simulink model "untitled"  (R2025b)
settings: Solver=ode1be  StartTime=0.0  StopTime=15  FixedStep=0.001  RelTol=1e-3
undefined symbols (not defined in the file): DiscIntNeverNeededParam, X, Y, Z
libraries: sm_lib x94, nesl_utility x30, fl_lib x14, ee_lib x5, simulink_extras x4, instrumentseriallib x4, etargetslib x3
(part 3 of 4)

== system untitled/Subsystem1/시스템 응답특성 ==
  MATLAB Function : MATLAB Function  TreatAsAtomicUnit=on
  감쇠비 : Display
  감쇠진동수 : Display
  고유진동수 : Display
  정착시간 : Display
  진동횟수 : Display
  wires:
  MATLAB Function/1(wn) -> 고유진동수/1
  MATLAB Function/3(wd) -> 감쇠진동수/1
  MATLAB Function/4(ts) -> 정착시간/1
  MATLAB Function/2(zeta) -> 감쇠비/1
  [cal_d] -> MATLAB Function/2(kd)
  [cal_p] -> MATLAB Function/1(kp)
  MATLAB Function/5(N) -> 진동횟수/1

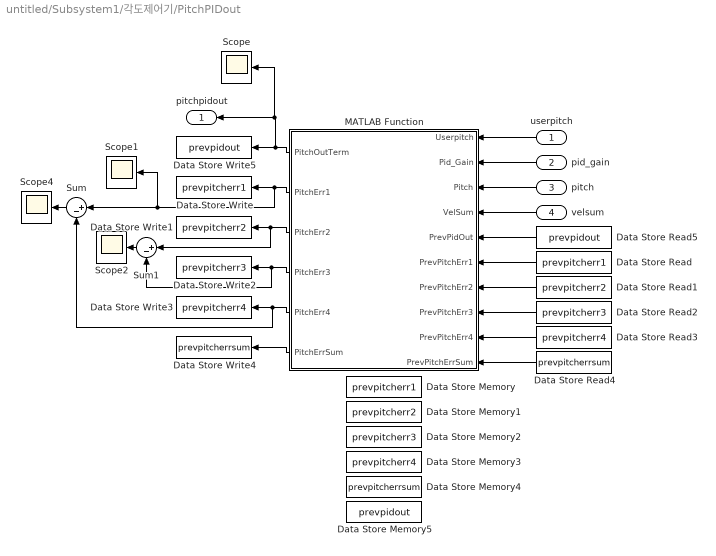
== system untitled/Subsystem1/각도제어기/PitchPIDout ==
  userpitch : Inport
  pid_gain : Inport  Port=2
  pitch : Inport  Port=3
  velsum : Inport  Port=4
  Data Store Memory : DataStoreMemory  DataStoreName=prevpitcherr1  WriteAfterWriteMsg=warning  ShowAdditionalParam=off
  Data Store Memory1 : DataStoreMemory  DataStoreName=prevpitcherr2  WriteAfterWriteMsg=warning  ShowAdditionalParam=off
  Data Store Memory2 : DataStoreMemory  DataStoreName=prevpitcherr3  WriteAfterWriteMsg=warning  ShowAdditionalParam=off
  Data Store Memory3 : DataStoreMemory  DataStoreName=prevpitcherr4  WriteAfterWriteMsg=warning  ShowAdditionalParam=off
  Data Store Memory4 : DataStoreMemory  DataStoreName=prevpitcherrsum  WriteAfterWriteMsg=warning  ShowAdditionalParam=off
  Data Store Memory5 : DataStoreMemory  DataStoreName=prevpidout  WriteAfterWriteMsg=warning  ShowAdditionalParam=off
  Data Store Read : DataStoreRead  DataStoreName=prevpitcherr1  IndexOptions=Index vector (dialog)  Indices=1  OutputSizes=1
  Data Store Read1 : DataStoreRead  DataStoreName=prevpitcherr2  IndexOptions=Index vector (dialog)  Indices=1  OutputSizes=1
  Data Store Read2 : DataStoreRead  DataStoreName=prevpitcherr3  IndexOptions=Index vector (dialog)  Indices=1  OutputSizes=1
  Data Store Read3 : DataStoreRead  DataStoreName=prevpitcherr4  IndexOptions=Index vector (dialog)  Indices=1  OutputSizes=1
  Data Store Read4 : DataStoreRead  DataStoreName=prevpitcherrsum  IndexOptions=Index vector (dialog)  Indices=1  OutputSizes=1
  Data Store Read5 : DataStoreRead  DataStoreName=prevpidout  IndexOptions=Index vector (dialog)  Indices=1  OutputSizes=1
  Data Store Write : DataStoreWrite  DataStoreName=prevpitcherr1  IndexOptions=Index vector (dialog)  Indices=1  OutputSizes=1
  Data Store Write1 : DataStoreWrite  DataStoreName=prevpitcherr2  IndexOptions=Index vector (dialog)  Indices=1  OutputSizes=1
  Data Store Write2 : DataStoreWrite  DataStoreName=prevpitcherr3  IndexOptions=Index vector (dialog)  Indices=1  OutputSizes=1
  Data Store Write3 : DataStoreWrite  DataStoreName=prevpitcherr4  IndexOptions=Index vector (dialog)  Indices=1  OutputSizes=1
  Data Store Write4 : DataStoreWrite  DataStoreName=prevpitcherrsum  IndexOptions=Index vector (dialog)  Indices=1  OutputSizes=1
  Data Store Write5 : DataStoreWrite  DataStoreName=prevpidout  IndexOptions=Index vector (dialog)  Indices=1  OutputSizes=1
  MATLAB Function : MATLAB Function  TreatAsAtomicUnit=on  SystemSampleTime=0.005
  Scope{,1..2,4} (4 alike) : Scope
      Scope settings: ActiveDisplayYMinimum=-0.020953586841830588  ActiveDisplayYMaximum=0.0054385268449779461  DataLoggingVariableName=ScopeData11
      Scope1 settings: ActiveDisplayYMinimum=-2.5668276523074756E-6  ActiveDisplayYMaximum=2.3101448870766709E-5  DataLoggingVariableName=ScopeData22
      Scope2 settings: ActiveDisplayYMinimum=-0.0010160045575017935  ActiveDisplayYMaximum=0.0011587189479117432  DataLoggingVariableName=ScopeData23
      Scope4 settings: ActiveDisplayYMinimum=-0.0018545960529793347  ActiveDisplayYMaximum=0.0021480135673250383  DataLoggingVariableName=ScopeData25
  Sum : Sum  Inputs=|+-
  Sum1 : Sum  Inputs=|+-
  pitchpidout : Outport
  wires:
  userpitch/1 -> MATLAB Function/1(Userpitch)
  pid_gain/1 -> MATLAB Function/2(Pid_Gain)
  pitch/1 -> MATLAB Function/3(Pitch)
  velsum/1 -> MATLAB Function/4(VelSum)
  Data Store Read5/1 -> MATLAB Function/5(PrevPidOut)
  Data Store Read/1 -> MATLAB Function/6(PrevPitchErr1)
  Data Store Read1/1 -> MATLAB Function/7(PrevPitchErr2)
  Data Store Read2/1 -> MATLAB Function/8(PrevPitchErr3)
  Data Store Read3/1 -> MATLAB Function/9(PrevPitchErr4)
  Data Store Read4/1 -> MATLAB Function/10(PrevPitchErrSum)
  MATLAB Function/1(PitchOutTerm) -> Scope/1, pitchpidout/1, Data Store Write5/1
  MATLAB Function/2(PitchErr1) -> Scope1/1, Sum/1, Data Store Write/1
  MATLAB Function/6(PitchErrSum) -> Data Store Write4/1
  MATLAB Function/3(PitchErr2) -> Sum1/1, Data Store Write1/1
  MATLAB Function/4(PitchErr3) -> Sum1/2, Data Store Write2/1
  MATLAB Function/5(PitchErr4) -> Sum/2, Data Store Write3/1
  Sum/1 -> Scope4/1
  Sum1/1 -> Scope2/1

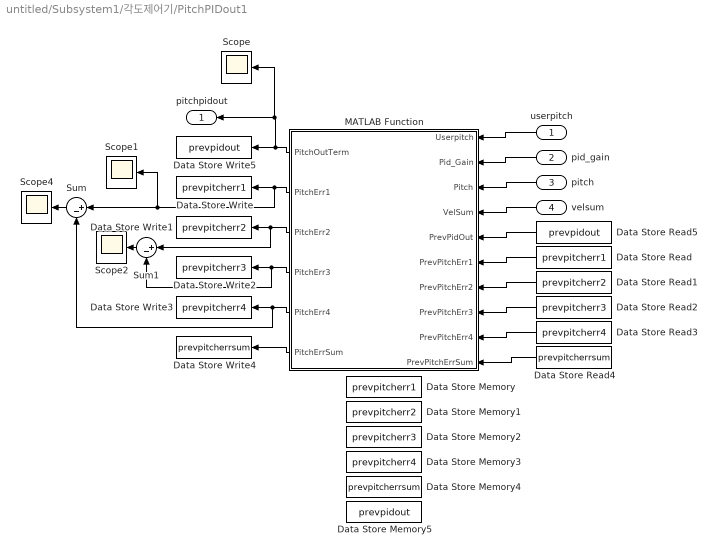
== system untitled/Subsystem1/각도제어기/PitchPIDout1 ==
  userpitch : Inport
  pid_gain : Inport  Port=2
  pitch : Inport  Port=3
  velsum : Inport  Port=4
  Data Store Memory : DataStoreMemory  DataStoreName=prevpitcherr1  WriteAfterWriteMsg=warning  ShowAdditionalParam=off
  Data Store Memory1 : DataStoreMemory  DataStoreName=prevpitcherr2  WriteAfterWriteMsg=warning  ShowAdditionalParam=off
  Data Store Memory2 : DataStoreMemory  DataStoreName=prevpitcherr3  WriteAfterWriteMsg=warning  ShowAdditionalParam=off
  Data Store Memory3 : DataStoreMemory  DataStoreName=prevpitcherr4  WriteAfterWriteMsg=warning  ShowAdditionalParam=off
  Data Store Memory4 : DataStoreMemory  DataStoreName=prevpitcherrsum  WriteAfterWriteMsg=warning  ShowAdditionalParam=off
  Data Store Memory5 : DataStoreMemory  DataStoreName=prevpidout  WriteAfterWriteMsg=warning  ShowAdditionalParam=off
  Data Store Read : DataStoreRead  DataStoreName=prevpitcherr1  IndexOptions=Index vector (dialog)  Indices=1  OutputSizes=1
  Data Store Read1 : DataStoreRead  DataStoreName=prevpitcherr2  IndexOptions=Index vector (dialog)  Indices=1  OutputSizes=1
  Data Store Read2 : DataStoreRead  DataStoreName=prevpitcherr3  IndexOptions=Index vector (dialog)  Indices=1  OutputSizes=1
  Data Store Read3 : DataStoreRead  DataStoreName=prevpitcherr4  IndexOptions=Index vector (dialog)  Indices=1  OutputSizes=1
  Data Store Read4 : DataStoreRead  DataStoreName=prevpitcherrsum  IndexOptions=Index vector (dialog)  Indices=1  OutputSizes=1
  Data Store Read5 : DataStoreRead  DataStoreName=prevpidout  IndexOptions=Index vector (dialog)  Indices=1  OutputSizes=1
  Data Store Write : DataStoreWrite  DataStoreName=prevpitcherr1  IndexOptions=Index vector (dialog)  Indices=1  OutputSizes=1
  Data Store Write1 : DataStoreWrite  DataStoreName=prevpitcherr2  IndexOptions=Index vector (dialog)  Indices=1  OutputSizes=1
  Data Store Write2 : DataStoreWrite  DataStoreName=prevpitcherr3  IndexOptions=Index vector (dialog)  Indices=1  OutputSizes=1
  Data Store Write3 : DataStoreWrite  DataStoreName=prevpitcherr4  IndexOptions=Index vector (dialog)  Indices=1  OutputSizes=1
  Data Store Write4 : DataStoreWrite  DataStoreName=prevpitcherrsum  IndexOptions=Index vector (dialog)  Indices=1  OutputSizes=1
  Data Store Write5 : DataStoreWrite  DataStoreName=prevpidout  IndexOptions=Index vector (dialog)  Indices=1  OutputSizes=1
  MATLAB Function : MATLAB Function  TreatAsAtomicUnit=on  SystemSampleTime=0.005
  Scope{,1..2,4} (4 alike) : Scope
      Scope settings: ActiveDisplayYMinimum=-0.020953586841830588  ActiveDisplayYMaximum=0.0054385268449779461  DataLoggingVariableName=ScopeData11
      Scope1 settings: ActiveDisplayYMinimum=-2.5668276523074756E-6  ActiveDisplayYMaximum=2.3101448870766709E-5  DataLoggingVariableName=ScopeData22
      Scope2 settings: ActiveDisplayYMinimum=-0.0010160045575017935  ActiveDisplayYMaximum=0.0011587189479117432  DataLoggingVariableName=ScopeData23
      Scope4 settings: ActiveDisplayYMinimum=-0.0018545960529793347  ActiveDisplayYMaximum=0.0021480135673250383  DataLoggingVariableName=ScopeData25
  Sum : Sum  Inputs=|+-
  Sum1 : Sum  Inputs=|+-
  pitchpidout : Outport
  wires:
  userpitch/1 -> MATLAB Function/1(Userpitch)
  pid_gain/1 -> MATLAB Function/2(Pid_Gain)
  pitch/1 -> MATLAB Function/3(Pitch)
  velsum/1 -> MATLAB Function/4(VelSum)
  Data Store Read5/1 -> MATLAB Function/5(PrevPidOut)
  Data Store Read/1 -> MATLAB Function/6(PrevPitchErr1)
  Data Store Read1/1 -> MATLAB Function/7(PrevPitchErr2)
  Data Store Read2/1 -> MATLAB Function/8(PrevPitchErr3)
  Data Store Read3/1 -> MATLAB Function/9(PrevPitchErr4)
  Data Store Read4/1 -> MATLAB Function/10(PrevPitchErrSum)
  MATLAB Function/1(PitchOutTerm) -> Scope/1, pitchpidout/1, Data Store Write5/1
  MATLAB Function/2(PitchErr1) -> Scope1/1, Sum/1, Data Store Write/1
  MATLAB Function/6(PitchErrSum) -> Data Store Write4/1
  MATLAB Function/3(PitchErr2) -> Sum1/1, Data Store Write1/1
  MATLAB Function/4(PitchErr3) -> Sum1/2, Data Store Write2/1
  MATLAB Function/5(PitchErr4) -> Sum/2, Data Store Write3/1
  Sum/1 -> Scope4/1
  Sum1/1 -> Scope2/1

== system untitled/Subsystem1/각도제어기/TargetPIDout ==
  TargetVel : Inport
  robot_vel : Inport  Port=2
  pid_gain : Inport  Port=3
  Data Store Memory : DataStoreMemory  DataStoreName=prevTargeterr1  WriteAfterWriteMsg=warning  ShowAdditionalParam=off
  Data Store Memory1 : DataStoreMemory  DataStoreName=prevTargeterr2  WriteAfterWriteMsg=warning  ShowAdditionalParam=off
  Data Store Memory2 : DataStoreMemory  DataStoreName=prevTargeterr3  WriteAfterWriteMsg=warning  ShowAdditionalParam=off
  Data Store Memory3 : DataStoreMemory  DataStoreName=prevTargeterr4  WriteAfterWriteMsg=warning  ShowAdditionalParam=off
  Data Store Memory4 : DataStoreMemory  DataStoreName=prevTargetErrSum  WriteAfterWriteMsg=warning  ShowAdditionalParam=off
  Data Store Memory5 : DataStoreMemory  DataStoreName=Prevpidout  WriteAfterWriteMsg=warning  ShowAdditionalParam=off
  Data Store Read : DataStoreRead  DataStoreName=prevTargeterr1  IndexOptions=Index vector (dialog)  Indices=1  OutputSizes=1
  Data Store Read1 : DataStoreRead  DataStoreName=prevTargeterr2  IndexOptions=Index vector (dialog)  Indices=1  OutputSizes=1
  Data Store Read2 : DataStoreRead  DataStoreName=prevTargeterr3  IndexOptions=Index vector (dialog)  Indices=1  OutputSizes=1
  Data Store Read3 : DataStoreRead  DataStoreName=prevTargeterr4  IndexOptions=Index vector (dialog)  Indices=1  OutputSizes=1
  Data Store Read4 : DataStoreRead  DataStoreName=prevTargetErrSum  IndexOptions=Index vector (dialog)  Indices=1  OutputSizes=1
  Data Store Read5 : DataStoreRead  DataStoreName=Prevpidout  IndexOptions=Index vector (dialog)  Indices=1  OutputSizes=1
  Data Store Write : DataStoreWrite  DataStoreName=prevTargeterr1  IndexOptions=Index vector (dialog)  Indices=1  OutputSizes=1
  Data Store Write1 : DataStoreWrite  DataStoreName=prevTargeterr2  IndexOptions=Index vector (dialog)  Indices=1  OutputSizes=1
  Data Store Write2 : DataStoreWrite  DataStoreName=prevTargeterr3  IndexOptions=Index vector (dialog)  Indices=1  OutputSizes=1
  Data Store Write3 : DataStoreWrite  DataStoreName=prevTargeterr4  IndexOptions=Index vector (dialog)  Indices=1  OutputSizes=1
  Data Store Write4 : DataStoreWrite  DataStoreName=prevTargetErrSum  IndexOptions=Index vector (dialog)  Indices=1  OutputSizes=1
  Data Store Write5 : DataStoreWrite  DataStoreName=Prevpidout  IndexOptions=Index vector (dialog)  Indices=1  OutputSizes=1
  MATLAB Function : MATLAB Function  TreatAsAtomicUnit=on  SystemSampleTime=0.005
  UserPitch : Outport
  wires:
  Data Store Read5/1 -> MATLAB Function/4(PrevPidOut)
  MATLAB Function/6(TargetErrSum) -> Data Store Write4/1
  Data Store Read3/1 -> MATLAB Function/8(PrevTargetErr4)
  MATLAB Function/4(TargetErr3) -> Data Store Write2/1
  Data Store Read1/1 -> MATLAB Function/6(PrevTargetErr2)
  MATLAB Function/2(TargetErr1) -> Data Store Write/1
  Data Store Read4/1 -> MATLAB Function/9(PrevYawErrSum)
  Data Store Read2/1 -> MATLAB Function/7(PrevTargetErr3)
  pid_gain/1 -> MATLAB Function/3(Pid_Gain)
  MATLAB Function/1(UserPitch) -> UserPitch/1, Data Store Write5/1
  MATLAB Function/3(TargetErr2) -> Data Store Write1/1
  Data Store Read/1 -> MATLAB Function/5(PrevTargetErr1)
  TargetVel/1 -> MATLAB Function/1(TargetVel)
  MATLAB Function/5(TargetErr4) -> Data Store Write3/1
  robot_vel/1 -> MATLAB Function/2(robot_vel)

== system untitled/Subsystem1/각도제어기/TargetPIDout1 ==
  TargetVel : Inport
  robot_vel : Inport  Port=2
  pid_gain : Inport  Port=3
  Data Store Memory : DataStoreMemory  DataStoreName=prevTargeterr1  WriteAfterWriteMsg=warning  ShowAdditionalParam=off
  Data Store Memory1 : DataStoreMemory  DataStoreName=prevTargeterr2  WriteAfterWriteMsg=warning  ShowAdditionalParam=off
  Data Store Memory2 : DataStoreMemory  DataStoreName=prevTargeterr3  WriteAfterWriteMsg=warning  ShowAdditionalParam=off
  Data Store Memory3 : DataStoreMemory  DataStoreName=prevTargeterr4  WriteAfterWriteMsg=warning  ShowAdditionalParam=off
  Data Store Memory4 : DataStoreMemory  DataStoreName=prevTargetErrSum  WriteAfterWriteMsg=warning  ShowAdditionalParam=off
  Data Store Memory5 : DataStoreMemory  DataStoreName=Prevpidout  WriteAfterWriteMsg=warning  ShowAdditionalParam=off
  Data Store Read : DataStoreRead  DataStoreName=prevTargeterr1  IndexOptions=Index vector (dialog)  Indices=1  OutputSizes=1
  Data Store Read1 : DataStoreRead  DataStoreName=prevTargeterr2  IndexOptions=Index vector (dialog)  Indices=1  OutputSizes=1
  Data Store Read2 : DataStoreRead  DataStoreName=prevTargeterr3  IndexOptions=Index vector (dialog)  Indices=1  OutputSizes=1
  Data Store Read3 : DataStoreRead  DataStoreName=prevTargeterr4  IndexOptions=Index vector (dialog)  Indices=1  OutputSizes=1
  Data Store Read4 : DataStoreRead  DataStoreName=prevTargetErrSum  IndexOptions=Index vector (dialog)  Indices=1  OutputSizes=1
  Data Store Read5 : DataStoreRead  DataStoreName=Prevpidout  IndexOptions=Index vector (dialog)  Indices=1  OutputSizes=1
  Data Store Write : DataStoreWrite  DataStoreName=prevTargeterr1  IndexOptions=Index vector (dialog)  Indices=1  OutputSizes=1
  Data Store Write1 : DataStoreWrite  DataStoreName=prevTargeterr2  IndexOptions=Index vector (dialog)  Indices=1  OutputSizes=1
  Data Store Write2 : DataStoreWrite  DataStoreName=prevTargeterr3  IndexOptions=Index vector (dialog)  Indices=1  OutputSizes=1
  Data Store Write3 : DataStoreWrite  DataStoreName=prevTargeterr4  IndexOptions=Index vector (dialog)  Indices=1  OutputSizes=1
  Data Store Write4 : DataStoreWrite  DataStoreName=prevTargetErrSum  IndexOptions=Index vector (dialog)  Indices=1  OutputSizes=1
  Data Store Write5 : DataStoreWrite  DataStoreName=Prevpidout  IndexOptions=Index vector (dialog)  Indices=1  OutputSizes=1
  MATLAB Function : MATLAB Function  TreatAsAtomicUnit=on  SystemSampleTime=0.005
  UserPitch : Outport
  wires:
  Data Store Read5/1 -> MATLAB Function/4(PrevPidOut)
  MATLAB Function/6(TargetErrSum) -> Data Store Write4/1
  Data Store Read3/1 -> MATLAB Function/8(PrevTargetErr4)
  MATLAB Function/4(TargetErr3) -> Data Store Write2/1
  Data Store Read1/1 -> MATLAB Function/6(PrevTargetErr2)
  MATLAB Function/2(TargetErr1) -> Data Store Write/1
  Data Store Read4/1 -> MATLAB Function/9(PrevYawErrSum)
  Data Store Read2/1 -> MATLAB Function/7(PrevTargetErr3)
  pid_gain/1 -> MATLAB Function/3(Pid_Gain)
  MATLAB Function/1(UserPitch) -> UserPitch/1, Data Store Write5/1
  MATLAB Function/3(TargetErr2) -> Data Store Write1/1
  Data Store Read/1 -> MATLAB Function/5(PrevTargetErr1)
  TargetVel/1 -> MATLAB Function/1(TargetVel)
  MATLAB Function/5(TargetErr4) -> Data Store Write3/1
  robot_vel/1 -> MATLAB Function/2(robot_vel)

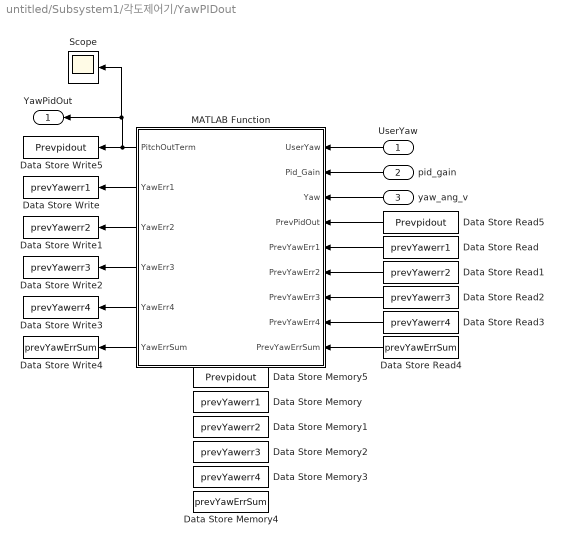
== system untitled/Subsystem1/각도제어기/YawPIDout ==
  UserYaw : Inport
  pid_gain : Inport  Port=2
  yaw_ang_v : Inport  Port=3
  Data Store Memory : DataStoreMemory  DataStoreName=prevYawerr1  WriteAfterWriteMsg=warning  ShowAdditionalParam=off
  Data Store Memory1 : DataStoreMemory  DataStoreName=prevYawerr2  WriteAfterWriteMsg=warning  ShowAdditionalParam=off
  Data Store Memory2 : DataStoreMemory  DataStoreName=prevYawerr3  WriteAfterWriteMsg=warning  ShowAdditionalParam=off
  Data Store Memory3 : DataStoreMemory  DataStoreName=prevYawerr4  WriteAfterWriteMsg=warning  ShowAdditionalParam=off
  Data Store Memory4 : DataStoreMemory  DataStoreName=prevYawErrSum  WriteAfterWriteMsg=warning  ShowAdditionalParam=off
  Data Store Memory5 : DataStoreMemory  DataStoreName=Prevpidout  WriteAfterWriteMsg=warning  ShowAdditionalParam=off
  Data Store Read : DataStoreRead  DataStoreName=prevYawerr1  IndexOptions=Index vector (dialog)  Indices=1  OutputSizes=1
  Data Store Read1 : DataStoreRead  DataStoreName=prevYawerr2  IndexOptions=Index vector (dialog)  Indices=1  OutputSizes=1
  Data Store Read2 : DataStoreRead  DataStoreName=prevYawerr3  IndexOptions=Index vector (dialog)  Indices=1  OutputSizes=1
  Data Store Read3 : DataStoreRead  DataStoreName=prevYawerr4  IndexOptions=Index vector (dialog)  Indices=1  OutputSizes=1
  Data Store Read4 : DataStoreRead  DataStoreName=prevYawErrSum  IndexOptions=Index vector (dialog)  Indices=1  OutputSizes=1
  Data Store Read5 : DataStoreRead  DataStoreName=Prevpidout  IndexOptions=Index vector (dialog)  Indices=1  OutputSizes=1
  Data Store Write : DataStoreWrite  DataStoreName=prevYawerr1  IndexOptions=Index vector (dialog)  Indices=1  OutputSizes=1
  Data Store Write1 : DataStoreWrite  DataStoreName=prevYawerr2  IndexOptions=Index vector (dialog)  Indices=1  OutputSizes=1
  Data Store Write2 : DataStoreWrite  DataStoreName=prevYawerr3  IndexOptions=Index vector (dialog)  Indices=1  OutputSizes=1
  Data Store Write3 : DataStoreWrite  DataStoreName=prevYawerr4  IndexOptions=Index vector (dialog)  Indices=1  OutputSizes=1
  Data Store Write4 : DataStoreWrite  DataStoreName=prevYawErrSum  IndexOptions=Index vector (dialog)  Indices=1  OutputSizes=1
  Data Store Write5 : DataStoreWrite  DataStoreName=Prevpidout  IndexOptions=Index vector (dialog)  Indices=1  OutputSizes=1
  MATLAB Function : MATLAB Function  TreatAsAtomicUnit=on  SystemSampleTime=0.005
  Scope : Scope
      settings: ActiveDisplayYMinimum=-0.13106550411433154  ActiveDisplayYMaximum=1.1795895370289842  DataLoggingVariableName=ScopeData15
  YawPidOut : Outport
  wires:
  Data Store Read5/1 -> MATLAB Function/4(PrevPidOut)
  MATLAB Function/6(YawErrSum) -> Data Store Write4/1
  Data Store Read3/1 -> MATLAB Function/8(PrevYawErr4)
  MATLAB Function/4(YawErr3) -> Data Store Write2/1
  Data Store Read1/1 -> MATLAB Function/6(PrevYawErr2)
  yaw_ang_v/1 -> MATLAB Function/3(Yaw)
  MATLAB Function/2(YawErr1) -> Data Store Write/1
  Data Store Read4/1 -> MATLAB Function/9(PrevYawErrSum)
  Data Store Read2/1 -> MATLAB Function/7(PrevYawErr3)
  pid_gain/1 -> MATLAB Function/2(Pid_Gain)
  MATLAB Function/1(PitchOutTerm) -> Scope/1, YawPidOut/1, Data Store Write5/1
  MATLAB Function/3(YawErr2) -> Data Store Write1/1
  Data Store Read/1 -> MATLAB Function/5(PrevYawErr1)
  UserYaw/1 -> MATLAB Function/1(UserYaw)
  MATLAB Function/5(YawErr4) -> Data Store Write3/1

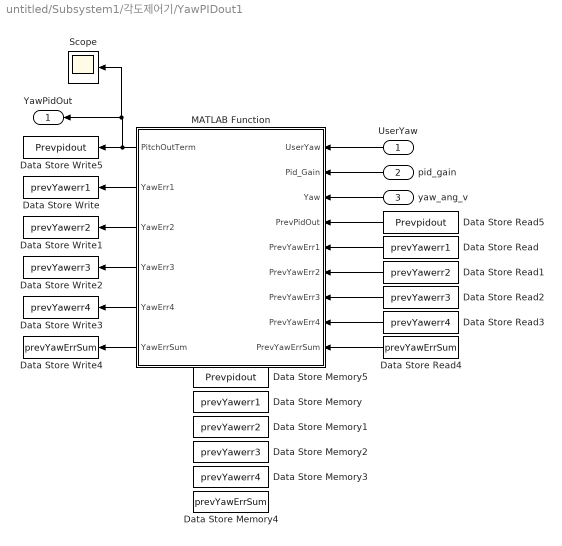
== system untitled/Subsystem1/각도제어기/YawPIDout1 ==
  UserYaw : Inport
  pid_gain : Inport  Port=2
  yaw_ang_v : Inport  Port=3
  Data Store Memory : DataStoreMemory  DataStoreName=prevYawerr1  WriteAfterWriteMsg=warning  ShowAdditionalParam=off
  Data Store Memory1 : DataStoreMemory  DataStoreName=prevYawerr2  WriteAfterWriteMsg=warning  ShowAdditionalParam=off
  Data Store Memory2 : DataStoreMemory  DataStoreName=prevYawerr3  WriteAfterWriteMsg=warning  ShowAdditionalParam=off
  Data Store Memory3 : DataStoreMemory  DataStoreName=prevYawerr4  WriteAfterWriteMsg=warning  ShowAdditionalParam=off
  Data Store Memory4 : DataStoreMemory  DataStoreName=prevYawErrSum  WriteAfterWriteMsg=warning  ShowAdditionalParam=off
  Data Store Memory5 : DataStoreMemory  DataStoreName=Prevpidout  WriteAfterWriteMsg=warning  ShowAdditionalParam=off
  Data Store Read : DataStoreRead  DataStoreName=prevYawerr1  IndexOptions=Index vector (dialog)  Indices=1  OutputSizes=1
  Data Store Read1 : DataStoreRead  DataStoreName=prevYawerr2  IndexOptions=Index vector (dialog)  Indices=1  OutputSizes=1
  Data Store Read2 : DataStoreRead  DataStoreName=prevYawerr3  IndexOptions=Index vector (dialog)  Indices=1  OutputSizes=1
  Data Store Read3 : DataStoreRead  DataStoreName=prevYawerr4  IndexOptions=Index vector (dialog)  Indices=1  OutputSizes=1
  Data Store Read4 : DataStoreRead  DataStoreName=prevYawErrSum  IndexOptions=Index vector (dialog)  Indices=1  OutputSizes=1
  Data Store Read5 : DataStoreRead  DataStoreName=Prevpidout  IndexOptions=Index vector (dialog)  Indices=1  OutputSizes=1
  Data Store Write : DataStoreWrite  DataStoreName=prevYawerr1  IndexOptions=Index vector (dialog)  Indices=1  OutputSizes=1
  Data Store Write1 : DataStoreWrite  DataStoreName=prevYawerr2  IndexOptions=Index vector (dialog)  Indices=1  OutputSizes=1
  Data Store Write2 : DataStoreWrite  DataStoreName=prevYawerr3  IndexOptions=Index vector (dialog)  Indices=1  OutputSizes=1
  Data Store Write3 : DataStoreWrite  DataStoreName=prevYawerr4  IndexOptions=Index vector (dialog)  Indices=1  OutputSizes=1
  Data Store Write4 : DataStoreWrite  DataStoreName=prevYawErrSum  IndexOptions=Index vector (dialog)  Indices=1  OutputSizes=1
  Data Store Write5 : DataStoreWrite  DataStoreName=Prevpidout  IndexOptions=Index vector (dialog)  Indices=1  OutputSizes=1
  MATLAB Function : MATLAB Function  TreatAsAtomicUnit=on  SystemSampleTime=0.005
  Scope : Scope
      settings: ActiveDisplayYMinimum=-0.13106550411433154  ActiveDisplayYMaximum=1.1795895370289842  DataLoggingVariableName=ScopeData15
  YawPidOut : Outport
  wires:
  Data Store Read5/1 -> MATLAB Function/4(PrevPidOut)
  MATLAB Function/6(YawErrSum) -> Data Store Write4/1
  Data Store Read3/1 -> MATLAB Function/8(PrevYawErr4)
  MATLAB Function/4(YawErr3) -> Data Store Write2/1
  Data Store Read1/1 -> MATLAB Function/6(PrevYawErr2)
  yaw_ang_v/1 -> MATLAB Function/3(Yaw)
  MATLAB Function/2(YawErr1) -> Data Store Write/1
  Data Store Read4/1 -> MATLAB Function/9(PrevYawErrSum)
  Data Store Read2/1 -> MATLAB Function/7(PrevYawErr3)
  pid_gain/1 -> MATLAB Function/2(Pid_Gain)
  MATLAB Function/1(PitchOutTerm) -> Scope/1, YawPidOut/1, Data Store Write5/1
  MATLAB Function/3(YawErr2) -> Data Store Write1/1
  Data Store Read/1 -> MATLAB Function/5(PrevYawErr1)
  UserYaw/1 -> MATLAB Function/1(UserYaw)
  MATLAB Function/5(YawErr4) -> Data Store Write3/1

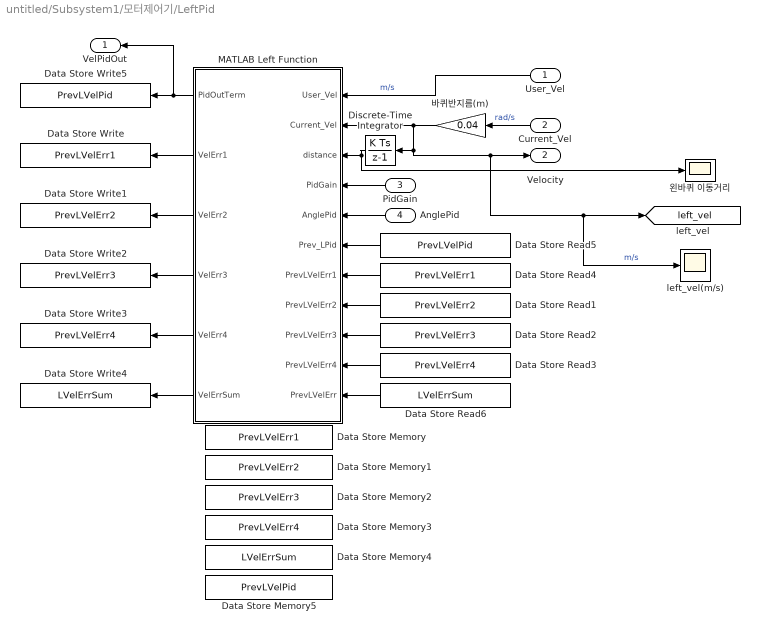
== system untitled/Subsystem1/모터제어기/LeftPid ==
  User_Vel : Inport
  Current_Vel : Inport  Port=2
  PidGain : Inport  Port=3
  AnglePid : Inport  Port=4
  Data Store Memory : DataStoreMemory  DataStoreName=PrevLVelErr1  WriteAfterWriteMsg=warning  ShowAdditionalParam=off
  Data Store Memory1 : DataStoreMemory  DataStoreName=PrevLVelErr2  WriteAfterWriteMsg=warning  ShowAdditionalParam=off
  Data Store Memory2 : DataStoreMemory  DataStoreName=PrevLVelErr3  WriteAfterWriteMsg=warning  ShowAdditionalParam=off
  Data Store Memory3 : DataStoreMemory  DataStoreName=PrevLVelErr4  WriteAfterWriteMsg=warning  ShowAdditionalParam=off
  Data Store Memory4 : DataStoreMemory  DataStoreName=LVelErrSum  WriteAfterWriteMsg=warning  ShowAdditionalParam=off
  Data Store Memory5 : DataStoreMemory  DataStoreName=PrevLVelPid  WriteAfterWriteMsg=warning  ShowAdditionalParam=off
  Data Store Read1 : DataStoreRead  DataStoreName=PrevLVelErr2  IndexOptions=Index vector (dialog)  Indices=1  OutputSizes=1
  Data Store Read2 : DataStoreRead  DataStoreName=PrevLVelErr3  IndexOptions=Index vector (dialog)  Indices=1  OutputSizes=1
  Data Store Read3 : DataStoreRead  DataStoreName=PrevLVelErr4  IndexOptions=Index vector (dialog)  Indices=1  OutputSizes=1
  Data Store Read4 : DataStoreRead  DataStoreName=PrevLVelErr1  IndexOptions=Index vector (dialog)  Indices=1  OutputSizes=1
  Data Store Read5 : DataStoreRead  DataStoreName=PrevLVelPid  IndexOptions=Index vector (dialog)  Indices=1  OutputSizes=1
  Data Store Read6 : DataStoreRead  DataStoreName=LVelErrSum  IndexOptions=Index vector (dialog)  Indices=1  OutputSizes=1
  Data Store Write : DataStoreWrite  DataStoreName=PrevLVelErr1  IndexOptions=Index vector (dialog)  Indices=1  OutputSizes=1
  Data Store Write1 : DataStoreWrite  DataStoreName=PrevLVelErr2  IndexOptions=Index vector (dialog)  Indices=1  OutputSizes=1
  Data Store Write2 : DataStoreWrite  DataStoreName=PrevLVelErr3  IndexOptions=Index vector (dialog)  Indices=1  OutputSizes=1
  Data Store Write3 : DataStoreWrite  DataStoreName=PrevLVelErr4  IndexOptions=Index vector (dialog)  Indices=1  OutputSizes=1
  Data Store Write4 : DataStoreWrite  DataStoreName=LVelErrSum  IndexOptions=Index vector (dialog)  Indices=1  OutputSizes=1
  Data Store Write5 : DataStoreWrite  DataStoreName=PrevLVelPid  IndexOptions=Index vector (dialog)  Indices=1  OutputSizes=1
  Discrete-Time Integrator : DiscreteIntegrator  SampleTime=0.005  ICPrevOutput=DiscIntNeverNeededParam  ICPrevScaledInput=DiscIntNeverNeededParam
  MATLAB Left Function : MATLAB Function  TreatAsAtomicUnit=on  SystemSampleTime=0.005
  left_vel(m/s) : Scope
      settings: ActiveDisplayYMinimum=-0.29402218772778749  ActiveDisplayYMaximum=0.33657759672028364  DataLoggingVariableName=ScopeData13
  바퀴반지름(m) : Gain  Gain=0.04
  왼바퀴 이동거리 : Scope
      settings: ActiveDisplayYMinimum=-0.013839886223825659  ActiveDisplayYMaximum=0.11819880478360369  DataLoggingVariableName=ScopeData9
  VelPidOut : Outport
  Velocity : Outport  Port=2
  tag scope: left_vel=global
  wires:
  User_Vel/1 -> MATLAB Left Function/1(User_Vel)  "m/s"
  PidGain/1 -> MATLAB Left Function/4(PidGain)
  AnglePid/1 -> MATLAB Left Function/5(AnglePid)
  Data Store Read4/1 -> MATLAB Left Function/7(PrevLVelErr1)
  Data Store Read2/1 -> MATLAB Left Function/9(PrevLVelErr3)
  MATLAB Left Function/6(VelErrSum) -> Data Store Write4/1
  MATLAB Left Function/5(VelErr4) -> Data Store Write3/1
  MATLAB Left Function/2(VelErr1) -> Data Store Write/1
  MATLAB Left Function/3(VelErr2) -> Data Store Write1/1
  MATLAB Left Function/4(VelErr3) -> Data Store Write2/1
  Data Store Read5/1 -> MATLAB Left Function/6(Prev_LPid)
  MATLAB Left Function/1(PidOutTerm) -> VelPidOut/1, Data Store Write5/1
  바퀴반지름(m)/1 -> MATLAB Left Function/2(Current_Vel), [left_vel], left_vel(m/s)/1, Velocity/1, Discrete-Time Integrator/1  "m/s"
  Current_Vel/1 -> 바퀴반지름(m)/1  "rad/s"
  Discrete-Time Integrator/1 -> 왼바퀴 이동거리/1, MATLAB Left Function/3(distance)
  Data Store Read1/1 -> MATLAB Left Function/8(PrevLVelErr2)
  Data Store Read3/1 -> MATLAB Left Function/10(PrevLVelErr4)
  Data Store Read6/1 -> MATLAB Left Function/11(PrevLVelErr)

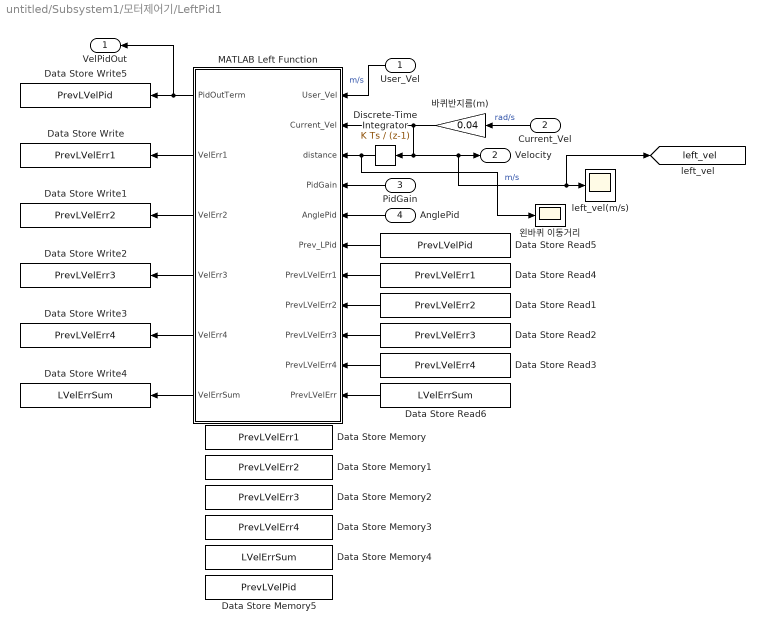
== system untitled/Subsystem1/모터제어기/LeftPid1 ==
  User_Vel : Inport
  Current_Vel : Inport  Port=2
  PidGain : Inport  Port=3
  AnglePid : Inport  Port=4
  Data Store Memory : DataStoreMemory  DataStoreName=PrevLVelErr1  WriteAfterWriteMsg=warning  ShowAdditionalParam=off
  Data Store Memory1 : DataStoreMemory  DataStoreName=PrevLVelErr2  WriteAfterWriteMsg=warning  ShowAdditionalParam=off
  Data Store Memory2 : DataStoreMemory  DataStoreName=PrevLVelErr3  WriteAfterWriteMsg=warning  ShowAdditionalParam=off
  Data Store Memory3 : DataStoreMemory  DataStoreName=PrevLVelErr4  WriteAfterWriteMsg=warning  ShowAdditionalParam=off
  Data Store Memory4 : DataStoreMemory  DataStoreName=LVelErrSum  WriteAfterWriteMsg=warning  ShowAdditionalParam=off
  Data Store Memory5 : DataStoreMemory  DataStoreName=PrevLVelPid  WriteAfterWriteMsg=warning  ShowAdditionalParam=off
  Data Store Read1 : DataStoreRead  DataStoreName=PrevLVelErr2  IndexOptions=Index vector (dialog)  Indices=1  OutputSizes=1
  Data Store Read2 : DataStoreRead  DataStoreName=PrevLVelErr3  IndexOptions=Index vector (dialog)  Indices=1  OutputSizes=1
  Data Store Read3 : DataStoreRead  DataStoreName=PrevLVelErr4  IndexOptions=Index vector (dialog)  Indices=1  OutputSizes=1
  Data Store Read4 : DataStoreRead  DataStoreName=PrevLVelErr1  IndexOptions=Index vector (dialog)  Indices=1  OutputSizes=1
  Data Store Read5 : DataStoreRead  DataStoreName=PrevLVelPid  IndexOptions=Index vector (dialog)  Indices=1  OutputSizes=1
  Data Store Read6 : DataStoreRead  DataStoreName=LVelErrSum  IndexOptions=Index vector (dialog)  Indices=1  OutputSizes=1
  Data Store Write : DataStoreWrite  DataStoreName=PrevLVelErr1  IndexOptions=Index vector (dialog)  Indices=1  OutputSizes=1
  Data Store Write1 : DataStoreWrite  DataStoreName=PrevLVelErr2  IndexOptions=Index vector (dialog)  Indices=1  OutputSizes=1
  Data Store Write2 : DataStoreWrite  DataStoreName=PrevLVelErr3  IndexOptions=Index vector (dialog)  Indices=1  OutputSizes=1
  Data Store Write3 : DataStoreWrite  DataStoreName=PrevLVelErr4  IndexOptions=Index vector (dialog)  Indices=1  OutputSizes=1
  Data Store Write4 : DataStoreWrite  DataStoreName=LVelErrSum  IndexOptions=Index vector (dialog)  Indices=1  OutputSizes=1
  Data Store Write5 : DataStoreWrite  DataStoreName=PrevLVelPid  IndexOptions=Index vector (dialog)  Indices=1  OutputSizes=1
  Discrete-Time Integrator : DiscreteIntegrator  SampleTime=0.005  ICPrevOutput=DiscIntNeverNeededParam  ICPrevScaledInput=DiscIntNeverNeededParam
  MATLAB Left Function : MATLAB Function  TreatAsAtomicUnit=on  SystemSampleTime=0.005
  left_vel(m/s) : Scope
      settings: ActiveDisplayYMinimum=-0.29402218772778749  ActiveDisplayYMaximum=0.33657759672028364  DataLoggingVariableName=ScopeData13
  바퀴반지름(m) : Gain  Gain=0.04
  왼바퀴 이동거리 : Scope
      settings: ActiveDisplayYMinimum=-0.013839886223825659  ActiveDisplayYMaximum=0.11819880478360369  DataLoggingVariableName=ScopeData9
  VelPidOut : Outport
  Velocity : Outport  Port=2
  tag scope: left_vel=global
  wires:
  User_Vel/1 -> MATLAB Left Function/1(User_Vel)  "m/s"
  PidGain/1 -> MATLAB Left Function/4(PidGain)
  AnglePid/1 -> MATLAB Left Function/5(AnglePid)
  Data Store Read4/1 -> MATLAB Left Function/7(PrevLVelErr1)
  Data Store Read2/1 -> MATLAB Left Function/9(PrevLVelErr3)
  MATLAB Left Function/6(VelErrSum) -> Data Store Write4/1
  MATLAB Left Function/5(VelErr4) -> Data Store Write3/1
  MATLAB Left Function/2(VelErr1) -> Data Store Write/1
  MATLAB Left Function/3(VelErr2) -> Data Store Write1/1
  MATLAB Left Function/4(VelErr3) -> Data Store Write2/1
  Data Store Read5/1 -> MATLAB Left Function/6(Prev_LPid)
  MATLAB Left Function/1(PidOutTerm) -> VelPidOut/1, Data Store Write5/1
  바퀴반지름(m)/1 -> MATLAB Left Function/2(Current_Vel), Discrete-Time Integrator/1, [left_vel], left_vel(m/s)/1, Velocity/1  "m/s"
  Current_Vel/1 -> 바퀴반지름(m)/1  "rad/s"
  Discrete-Time Integrator/1 -> 왼바퀴 이동거리/1, MATLAB Left Function/3(distance)
  Data Store Read1/1 -> MATLAB Left Function/8(PrevLVelErr2)
  Data Store Read3/1 -> MATLAB Left Function/10(PrevLVelErr4)
  Data Store Read6/1 -> MATLAB Left Function/11(PrevLVelErr)

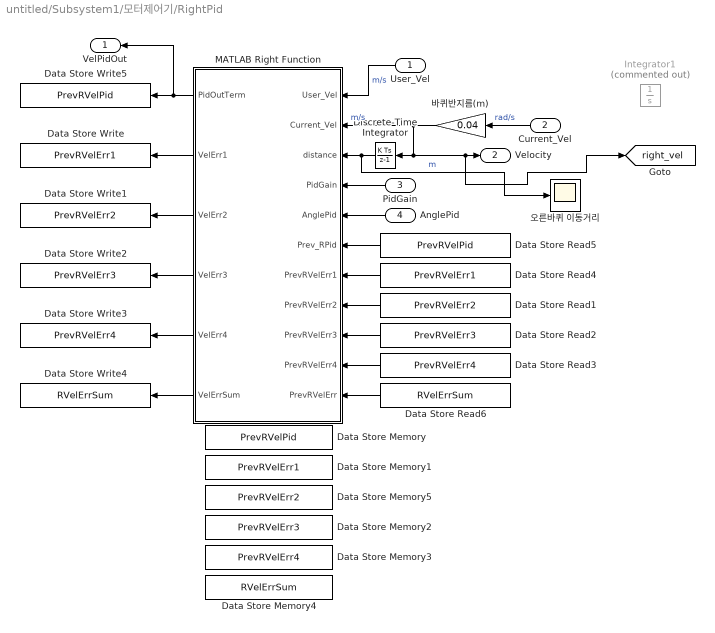
== system untitled/Subsystem1/모터제어기/RightPid ==
  User_Vel : Inport
  Current_Vel : Inport  Port=2
  PidGain : Inport  Port=3
  AnglePid : Inport  Port=4
  Data Store Memory : DataStoreMemory  DataStoreName=PrevRVelPid  WriteAfterWriteMsg=warning  ShowAdditionalParam=off
  Data Store Memory1 : DataStoreMemory  DataStoreName=PrevRVelErr1  WriteAfterWriteMsg=warning  ShowAdditionalParam=off
  Data Store Memory2 : DataStoreMemory  DataStoreName=PrevRVelErr3  WriteAfterWriteMsg=warning  ShowAdditionalParam=off
  Data Store Memory3 : DataStoreMemory  DataStoreName=PrevRVelErr4  WriteAfterWriteMsg=warning  ShowAdditionalParam=off
  Data Store Memory4 : DataStoreMemory  DataStoreName=RVelErrSum  WriteAfterWriteMsg=warning  ShowAdditionalParam=off
  Data Store Memory5 : DataStoreMemory  DataStoreName=PrevRVelErr2  WriteAfterWriteMsg=warning  ShowAdditionalParam=off
  Data Store Read1 : DataStoreRead  DataStoreName=PrevRVelErr2  IndexOptions=Index vector (dialog)  Indices=1  OutputSizes=1
  Data Store Read2 : DataStoreRead  DataStoreName=PrevRVelErr3  IndexOptions=Index vector (dialog)  Indices=1  OutputSizes=1
  Data Store Read3 : DataStoreRead  DataStoreName=PrevRVelErr4  IndexOptions=Index vector (dialog)  Indices=1  OutputSizes=1
  Data Store Read4 : DataStoreRead  DataStoreName=PrevRVelErr1  IndexOptions=Index vector (dialog)  Indices=1  OutputSizes=1
  Data Store Read5 : DataStoreRead  DataStoreName=PrevRVelPid  IndexOptions=Index vector (dialog)  Indices=1  OutputSizes=1
  Data Store Read6 : DataStoreRead  DataStoreName=RVelErrSum  IndexOptions=Index vector (dialog)  Indices=1  OutputSizes=1
  Data Store Write : DataStoreWrite  DataStoreName=PrevRVelErr1  IndexOptions=Index vector (dialog)  Indices=1  OutputSizes=1
  Data Store Write1 : DataStoreWrite  DataStoreName=PrevRVelErr2  IndexOptions=Index vector (dialog)  Indices=1  OutputSizes=1
  Data Store Write2 : DataStoreWrite  DataStoreName=PrevRVelErr3  IndexOptions=Index vector (dialog)  Indices=1  OutputSizes=1
  Data Store Write3 : DataStoreWrite  DataStoreName=PrevRVelErr4  IndexOptions=Index vector (dialog)  Indices=1  OutputSizes=1
  Data Store Write4 : DataStoreWrite  DataStoreName=RVelErrSum  IndexOptions=Index vector (dialog)  Indices=1  OutputSizes=1
  Data Store Write5 : DataStoreWrite  DataStoreName=PrevRVelPid  IndexOptions=Index vector (dialog)  Indices=1  OutputSizes=1
  Discrete-Time Integrator : DiscreteIntegrator  SampleTime=0.005  ICPrevOutput=DiscIntNeverNeededParam  ICPrevScaledInput=DiscIntNeverNeededParam
  Integrator1 : Integrator  Commented=on
  MATLAB Right Function : MATLAB Function  TreatAsAtomicUnit=on  SystemSampleTime=0.005
  바퀴반지름(m) : Gain  Gain=0.04
  오른바퀴 이동거리 : Scope
      settings: ActiveDisplayYMinimum=-0.061281693302219581  ActiveDisplayYMaximum=0.37221437509263816  DataLoggingVariableName=ScopeData9
  VelPidOut : Outport
  Velocity : Outport  Port=2
  tag scope: right_vel=global
  wires:
  User_Vel/1 -> MATLAB Right Function/1(User_Vel)  "m/s"
  PidGain/1 -> MATLAB Right Function/4(PidGain)
  AnglePid/1 -> MATLAB Right Function/5(AnglePid)
  Data Store Read4/1 -> MATLAB Right Function/7(PrevRVelErr1)
  Data Store Read2/1 -> MATLAB Right Function/9(PrevRVelErr3)
  MATLAB Right Function/6(VelErrSum) -> Data Store Write4/1
  MATLAB Right Function/5(VelErr4) -> Data Store Write3/1
  MATLAB Right Function/2(VelErr1) -> Data Store Write/1
  MATLAB Right Function/3(VelErr2) -> Data Store Write1/1
  MATLAB Right Function/4(VelErr3) -> Data Store Write2/1
  Data Store Read5/1 -> MATLAB Right Function/6(Prev_RPid)
  MATLAB Right Function/1(PidOutTerm) -> VelPidOut/1, Data Store Write5/1
  바퀴반지름(m)/1 -> MATLAB Right Function/2(Current_Vel), Discrete-Time Integrator/1, [right_vel], Velocity/1  "m/s"
  Current_Vel/1 -> 바퀴반지름(m)/1  "rad/s"
  Discrete-Time Integrator/1 -> 오른바퀴 이동거리/1, MATLAB Right Function/3(distance)  "m"
  Data Store Read1/1 -> MATLAB Right Function/8(PrevRVelErr2)
  Data Store Read3/1 -> MATLAB Right Function/10(PrevRVelErr4)
  Data Store Read6/1 -> MATLAB Right Function/11(PrevRVelErr)

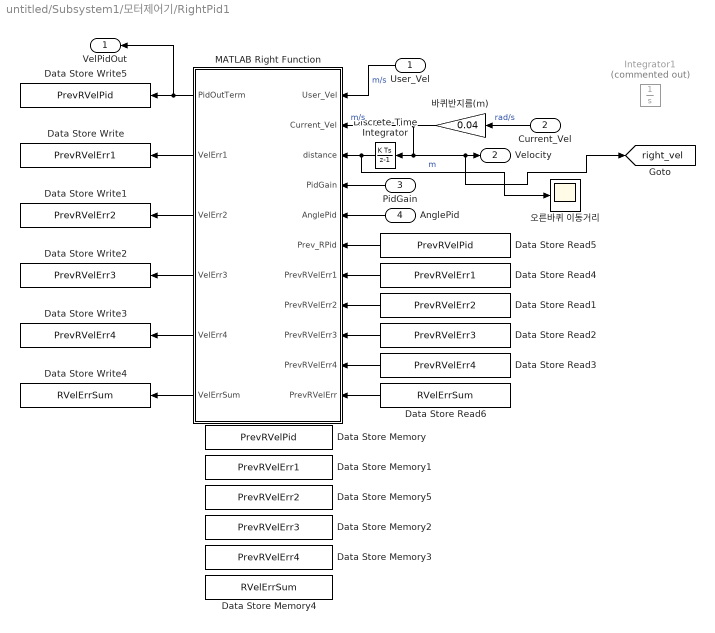
== system untitled/Subsystem1/모터제어기/RightPid1 ==
  User_Vel : Inport
  Current_Vel : Inport  Port=2
  PidGain : Inport  Port=3
  AnglePid : Inport  Port=4
  Data Store Memory : DataStoreMemory  DataStoreName=PrevRVelPid  WriteAfterWriteMsg=warning  ShowAdditionalParam=off
  Data Store Memory1 : DataStoreMemory  DataStoreName=PrevRVelErr1  WriteAfterWriteMsg=warning  ShowAdditionalParam=off
  Data Store Memory2 : DataStoreMemory  DataStoreName=PrevRVelErr3  WriteAfterWriteMsg=warning  ShowAdditionalParam=off
  Data Store Memory3 : DataStoreMemory  DataStoreName=PrevRVelErr4  WriteAfterWriteMsg=warning  ShowAdditionalParam=off
  Data Store Memory4 : DataStoreMemory  DataStoreName=RVelErrSum  WriteAfterWriteMsg=warning  ShowAdditionalParam=off
  Data Store Memory5 : DataStoreMemory  DataStoreName=PrevRVelErr2  WriteAfterWriteMsg=warning  ShowAdditionalParam=off
  Data Store Read1 : DataStoreRead  DataStoreName=PrevRVelErr2  IndexOptions=Index vector (dialog)  Indices=1  OutputSizes=1
  Data Store Read2 : DataStoreRead  DataStoreName=PrevRVelErr3  IndexOptions=Index vector (dialog)  Indices=1  OutputSizes=1
  Data Store Read3 : DataStoreRead  DataStoreName=PrevRVelErr4  IndexOptions=Index vector (dialog)  Indices=1  OutputSizes=1
  Data Store Read4 : DataStoreRead  DataStoreName=PrevRVelErr1  IndexOptions=Index vector (dialog)  Indices=1  OutputSizes=1
  Data Store Read5 : DataStoreRead  DataStoreName=PrevRVelPid  IndexOptions=Index vector (dialog)  Indices=1  OutputSizes=1
  Data Store Read6 : DataStoreRead  DataStoreName=RVelErrSum  IndexOptions=Index vector (dialog)  Indices=1  OutputSizes=1
  Data Store Write : DataStoreWrite  DataStoreName=PrevRVelErr1  IndexOptions=Index vector (dialog)  Indices=1  OutputSizes=1
  Data Store Write1 : DataStoreWrite  DataStoreName=PrevRVelErr2  IndexOptions=Index vector (dialog)  Indices=1  OutputSizes=1
  Data Store Write2 : DataStoreWrite  DataStoreName=PrevRVelErr3  IndexOptions=Index vector (dialog)  Indices=1  OutputSizes=1
  Data Store Write3 : DataStoreWrite  DataStoreName=PrevRVelErr4  IndexOptions=Index vector (dialog)  Indices=1  OutputSizes=1
  Data Store Write4 : DataStoreWrite  DataStoreName=RVelErrSum  IndexOptions=Index vector (dialog)  Indices=1  OutputSizes=1
  Data Store Write5 : DataStoreWrite  DataStoreName=PrevRVelPid  IndexOptions=Index vector (dialog)  Indices=1  OutputSizes=1
  Discrete-Time Integrator : DiscreteIntegrator  SampleTime=0.005  ICPrevOutput=DiscIntNeverNeededParam  ICPrevScaledInput=DiscIntNeverNeededParam
  Integrator1 : Integrator  Commented=on
  MATLAB Right Function : MATLAB Function  TreatAsAtomicUnit=on  SystemSampleTime=0.005
  바퀴반지름(m) : Gain  Gain=0.04
  오른바퀴 이동거리 : Scope
      settings: ActiveDisplayYMinimum=-0.061281693302219581  ActiveDisplayYMaximum=0.37221437509263816  DataLoggingVariableName=ScopeData9
  VelPidOut : Outport
  Velocity : Outport  Port=2
  tag scope: right_vel=global
  wires:
  User_Vel/1 -> MATLAB Right Function/1(User_Vel)  "m/s"
  PidGain/1 -> MATLAB Right Function/4(PidGain)
  AnglePid/1 -> MATLAB Right Function/5(AnglePid)
  Data Store Read4/1 -> MATLAB Right Function/7(PrevRVelErr1)
  Data Store Read2/1 -> MATLAB Right Function/9(PrevRVelErr3)
  MATLAB Right Function/6(VelErrSum) -> Data Store Write4/1
  MATLAB Right Function/5(VelErr4) -> Data Store Write3/1
  MATLAB Right Function/2(VelErr1) -> Data Store Write/1
  MATLAB Right Function/3(VelErr2) -> Data Store Write1/1
  MATLAB Right Function/4(VelErr3) -> Data Store Write2/1
  Data Store Read5/1 -> MATLAB Right Function/6(Prev_RPid)
  MATLAB Right Function/1(PidOutTerm) -> VelPidOut/1, Data Store Write5/1
  바퀴반지름(m)/1 -> MATLAB Right Function/2(Current_Vel), Discrete-Time Integrator/1, [right_vel], Velocity/1  "m/s"
  Current_Vel/1 -> 바퀴반지름(m)/1  "rad/s"
  Discrete-Time Integrator/1 -> 오른바퀴 이동거리/1, MATLAB Right Function/3(distance)  "m"
  Data Store Read1/1 -> MATLAB Right Function/8(PrevRVelErr2)
  Data Store Read3/1 -> MATLAB Right Function/10(PrevRVelErr4)
  Data Store Read6/1 -> MATLAB Right Function/11(PrevRVelErr)

== system untitled/Subsystem1/물리세계(땅, 로봇)/Subsystem ==
  In1 : Inport
  Trigger : TriggerPort  TriggerType=function-call  VariantControl=(inherit)  PortDimensions=1
  Byte Pack : etargetslib/Byte Pack  datatypes={'single'}  byteAlign=1
  Serial Send : instrumentseriallib/Serial Send  Priority=1  PortSel=COM13  Port=COM13  ComPort=COM13  Header=[]  Terminator=<none>  CustomTerminator=[]  EnableBlockingMode=off  SimulateUsing=Interpreted execution  BlockInModel=on  aMode=1
      settings: LibrarySourceBlock=embeddedtargetslib/Host Communication/Serial Send
  wires:
  Byte Pack/1 -> Serial Send/1
  In1/1 -> Byte Pack/1

== system untitled/Subsystem1/물리세계(땅, 로봇)/Subsystem1 ==
  In1 : Inport
  Trigger : TriggerPort  VariantControl=(inherit)  PortDimensions=1
  Byte Pack : etargetslib/Byte Pack  datatypes={'single'}  byteAlign=1
  Serial Send : instrumentseriallib/Serial Send  Priority=1  PortSel=COM13  Port=COM13  ComPort=COM13  Header=[]  Terminator=<none>  CustomTerminator=[]  EnableBlockingMode=on  SimulateUsing=Interpreted execution  BlockInModel=on  aMode=1
      settings: LibrarySourceBlock=embeddedtargetslib/Host Communication/Serial Send
  wires:
  Byte Pack/1 -> Serial Send/1
  In1/1 -> Byte Pack/1

== matlab function untitled/Subsystem1/물리세계(땅, 로봇)/MATLAB Function ==
  data: t input; force output
function force = fcn(t)
% t: 현재 시뮬레이션 시간 (입력)
% force: 출력할 외력 (N)

% 1초 지남(t >= 1) 그리고 2초가 되기 전(t <= 2)까지 0.1N 출력
if (t >= 2.0) && (t <= 2.1)
    force = 1.5;
else
    force = 0.0;
end

== matlab function untitled/Subsystem1/물리세계(땅, 로봇)/MATLAB Function1 ==
  data: t input; hip_deg output; knee_deg output
function [hip_deg, knee_deg] = fcn(t)
    % t: 현재 시뮬레이션 시간
    
    % 설정값
    delay = 1.0;      % 시작 전 대기 시간 (1초)
    end_time = 5.0;   % 동작이 끝나는 시간 (5초)
    motion_duration = end_time - delay; % 실제 동작 시간 (4초)
    half_duration = motion_duration / 2; % 굽히는 데 걸리는 시간 (2초)
    
    % 목표 각도 (최대로 굽혔을 때)
    hip_limit = 60;
    knee_limit = -106.36;
    
    if t < delay
        % 1단계: 1초 전에는 0도 유지
        ratio = 0;
        
    elseif t < (delay + half_duration)
        % 2단계: 1초 ~ 3초 동안 서서히 굽힘 (0 -> 1)
        ratio = (t - delay) / half_duration;
        
    elseif t < end_time
        % 3단계: 3초 ~ 5초 동안 서서히 폄 (1 -> 0)
        ratio = 1 - (t - (delay + half_duration)) / half_duration;
        
    else
        % 4단계: 5초 이후에는 다시 0도 고정
        ratio = 0;
    end
    
    % 최종 각도 계산
    hip_deg = hip_limit * ratio;
    knee_deg = knee_limit * ratio;
end

== matlab function untitled/Subsystem1/각도제어기/TargetPIDout/MATLAB Function ==
  data: UserPitch output; TargetErr1 output; TargetErr2 output; TargetErr3 output; TargetErr4 output; TargetErrSum output; TargetVel input; robot_vel input; Pid_Gain input; PrevPidOut input; PrevTargetErr1 input; PrevTargetErr2 input; PrevTargetErr3 input; PrevTargetErr4 input; PrevYawErrSum input
function [UserPitch, TargetErr1, TargetErr2, TargetErr3, TargetErr4, TargetErrSum] = ... %출력
fcn(TargetVel, robot_vel, Pid_Gain, PrevPidOut, PrevTargetErr1,...                  %입력
PrevTargetErr2, PrevTargetErr3, PrevTargetErr4, PrevYawErrSum)

tp = Pid_Gain(1);
ti = Pid_Gain(2);
td = Pid_Gain(3);

TargetErrSum = PrevYawErrSum;
TargetErr4 = PrevTargetErr4;
TargetErr3 = PrevTargetErr3;
TargetErr2 = PrevTargetErr2;
TargetErr1 = PrevTargetErr1;

%if(next_pitch > 30)
%    next_pitch = 30;
%elseif(next_pitch < -30)
%    next_pitch = -30;
%end

%TargetErrSum = TargetErrSum - TargetErr4;
TargetErr4 = TargetErr3;
TargetErr3 = TargetErr2;
TargetErr2 = TargetErr1;
TargetErr1 = TargetVel - robot_vel;
TargetErrSum = TargetErrSum + TargetErr1;

pid_p = tp*TargetErr1;
pid_i = ti*TargetErrSum;
pid_d = td*((TargetErr1 - TargetErr4)/0.005 + 2*(TargetErr2 - TargetErr3)/0.005);

UserPitch = pid_p + pid_i + pid_d; %단위: rad(라디안은 무차원임)

end

%5도를 유지하는 상황에서 robot_vel이 빨라지면 UserPitch는 음수가 됨.
%그럼 피치pid에서의 pid값이 음수가 되서 모터는 앞으로 가속함. 앞으로 가속하면
%로봇이 세워져서 robot_vel이 작아짐. 그럼 UserPitch는 양수가 됨. 그럼 피치pid에서
%pid값이 양수가 되서 뒤로 힘을 줘서 빨라짐. 이런 방식으로 로봇속도(robot_vel)는
%TargetPitch가 0이 아닐때 등속운동을 하게됨. 
%또한 TargetPitch가 0이고 외력을 받았을때 반대방향으로 움직일려고 해서 멈추게 됨.

== matlab function untitled/Subsystem1/시스템 응답특성/MATLAB Function ==
  data: kp input; wn output; kd input; zeta output; wd output; ts output; N output
function [wn, zeta, wd, ts, N] = fcn(kp, kd)

m = 0.5;      % 질량 (kg)
g = 9.81;     % 중력가속도 (m/s^2)
L = 0.11;      % 무게중심까지의 거리 (m)
J = m * L^2;  % 관성 모멘트 (kg*m^2)
b = 0.01;     % 시스템 마찰 계수 (실험치)


% 2. 계산 수행
A = (b + kd) / J;
B = (kp - m*g*L) / J;

wn = sqrt(complex(B));
zeta = A / (2 * wn);
wd = wn * sqrt(complex(1 - zeta^2));
ts = 4 / (zeta * wn);
N = (2 * sqrt(complex(1 - zeta^2))) / (pi * zeta);

end

== matlab function untitled/Subsystem1/각도제어기/MATLAB Function ==
  data: kp input; wn output; kd input; zeta output; wd output; ts output; N output
function [wn, zeta, wd, ts, N] = fcn(kp, kd)

m = 1;      % 질량 (kg)
g = 9.81;     % 중력가속도 (m/s^2)
L = 0.16;      % 무게중심까지의 거리 (m)
J = m * L^2;  % 관성 모멘트 (kg*m^2)
b = 0.03;     % 시스템 마찰 계수 (실험치)


% 2. 계산 수행
A = (b + kd) / J;
B = (kp - m*g*L) / J;

wn = sqrt(complex(B));
zeta = A / (2 * wn);
wd = wn * sqrt(complex(1 - zeta^2));
ts = 4 / (zeta * wn);
N = (2 * sqrt(complex(1 - zeta^2))) / (pi * zeta);

end

== matlab function untitled/Subsystem1/각도제어기/PitchPIDout1/MATLAB Function ==
  data: PitchOutTerm output; PitchErr1 output; PitchErr2 output; PitchErr3 output; PitchErr4 output; PitchErrSum output; Userpitch input; Pid_Gain input; Pitch input; VelSum input; PrevPidOut input; PrevPitchErr1 input; PrevPitchErr2 input; PrevPitchErr3 input; PrevPitchErr4 input; PrevPitchErrSum input
function [PitchOutTerm, PitchErr1, PitchErr2, PitchErr3, PitchErr4, PitchErrSum] = ... %출력
fcn(Userpitch, Pid_Gain, Pitch, VelSum, PrevPidOut, PrevPitchErr1,...                  %입력
PrevPitchErr2, PrevPitchErr3, PrevPitchErr4, PrevPitchErrSum)

kp = Pid_Gain(1);
ki = Pid_Gain(2);
kd = Pid_Gain(3);

PitchErrSum = PrevPitchErrSum;
PitchErr4 = PrevPitchErr4;
PitchErr3 = PrevPitchErr3;
PitchErr2 = PrevPitchErr2;
PitchErr1 = PrevPitchErr1;

%next_pitch = -(VelSum/90) + Userpitch;

%if(next_pitch > 30)
%    next_pitch = 30;
%elseif(next_pitch < -30)
%    next_pitch = -30;
%end

%PitchErrSum = PitchErrSum - PitchErr4;
PitchErr4 = PitchErr3;%이이이전오차
PitchErr3 = PitchErr2;%이이전오차
PitchErr2 = PitchErr1;%이전오차
PitchErr1 = Userpitch - Pitch;%현재오차
PitchErrSum = PitchErrSum + PitchErr1;

pid_p = kp*PitchErr1;%비례
pid_i = ki*(PitchErrSum);%적분
pid_d = kd*((PitchErr1 - PitchErr4)/0.005 + 2*(PitchErr2 - PitchErr3)/0.005);%미분

PitchOutTerm = pid_p + pid_i + pid_d; %단위: rad(라디안은 무차원임)
%PitchOutTerm = PrevPidOut + pid_p + pid_i + pid_d;
end

== matlab function untitled/Subsystem1/물리세계(땅, 로봇)/MATLAB Function3 ==
  data: v_in input; v_out output
function v_out = fcn(v_in)
    v_out = zeros(6,1);
    for i = 1:6
        % 통신 꼬임으로 인한 NaN이나 무한대 값이면 0V로 무시
        if isnan(v_in(i)) || isinf(v_in(i))
            v_out(i) = 0;
        % 정상 값이지만 너무 크면 배터리 한계인 +-20V로 강제 컷오프
        elseif v_in(i) > 10
            v_out(i) = 10;
        elseif v_in(i) < -10
            v_out(i) = -10;
        else
            v_out(i) = v_in(i);
        end
    end
end

== matlab function untitled/Subsystem1/각도제어기/TargetPIDout1/MATLAB Function ==
  data: UserPitch output; TargetErr1 output; TargetErr2 output; TargetErr3 output; TargetErr4 output; TargetErrSum output; TargetVel input; robot_vel input; Pid_Gain input; PrevPidOut input; PrevTargetErr1 input; PrevTargetErr2 input; PrevTargetErr3 input; PrevTargetErr4 input; PrevYawErrSum input
function [UserPitch, TargetErr1, TargetErr2, TargetErr3, TargetErr4, TargetErrSum] = ... %출력
fcn(TargetVel, robot_vel, Pid_Gain, PrevPidOut, PrevTargetErr1,...                  %입력
PrevTargetErr2, PrevTargetErr3, PrevTargetErr4, PrevYawErrSum)

tp = Pid_Gain(1);
ti = Pid_Gain(2);
td = Pid_Gain(3);

TargetErrSum = PrevYawErrSum;
TargetErr4 = PrevTargetErr4;
TargetErr3 = PrevTargetErr3;
TargetErr2 = PrevTargetErr2;
TargetErr1 = PrevTargetErr1;

%if(next_pitch > 30)
%    next_pitch = 30;
%elseif(next_pitch < -30)
%    next_pitch = -30;
%end

%TargetErrSum = TargetErrSum - TargetErr4;
TargetErr4 = TargetErr3;
TargetErr3 = TargetErr2;
TargetErr2 = TargetErr1;
TargetErr1 = TargetVel - robot_vel;
TargetErrSum = TargetErrSum + TargetErr1;

pid_p = tp*TargetErr1;
pid_i = ti*TargetErrSum;
pid_d = td*((TargetErr1 - TargetErr4)/0.005 + 2*(TargetErr2 - TargetErr3)/0.005);

UserPitch = pid_p + pid_i + pid_d; %단위: rad(라디안은 무차원임)

end

%5도를 유지하는 상황에서 robot_vel이 빨라지면 UserPitch는 음수가 됨.
%그럼 피치pid에서의 pid값이 음수가 되서 모터는 앞으로 가속함. 앞으로 가속하면
%로봇이 세워져서 robot_vel이 작아짐. 그럼 UserPitch는 양수가 됨. 그럼 피치pid에서
%pid값이 양수가 되서 뒤로 힘을 줘서 빨라짐. 이런 방식으로 로봇속도(robot_vel)는
%TargetPitch가 0이 아닐때 등속운동을 하게됨. 
%또한 TargetPitch가 0이고 외력을 받았을때 반대방향으로 움직일려고 해서 멈추게 됨.

== matlab function untitled/Subsystem1/각도제어기/YawPIDout1/MATLAB Function ==
  data: PitchOutTerm output; YawErr1 output; YawErr2 output; YawErr3 output; YawErr4 output; YawErrSum output; UserYaw input; Pid_Gain input; Yaw input; PrevPidOut input; PrevYawErr1 input; PrevYawErr2 input; PrevYawErr3 input; PrevYawErr4 input; PrevYawErrSum input
function [PitchOutTerm, YawErr1, YawErr2, YawErr3, YawErr4, YawErrSum] = ... %출력
fcn(UserYaw, Pid_Gain, Yaw, PrevPidOut, PrevYawErr1,...                  %입력
PrevYawErr2, PrevYawErr3, PrevYawErr4, PrevYawErrSum)

kp = Pid_Gain(1);
ki = Pid_Gain(2);
kd = Pid_Gain(3);

YawErrSum = PrevYawErrSum;
YawErr4 = PrevYawErr4;
YawErr3 = PrevYawErr3;
YawErr2 = PrevYawErr2;
YawErr1 = PrevYawErr1;

%if(next_pitch > 30)
%    next_pitch = 30;
%elseif(next_pitch < -30)
%    next_pitch = -30;
%end

YawErrSum = YawErrSum - YawErr4;
YawErr4 = YawErr3;
YawErr3 = YawErr2;
YawErr2 = YawErr1;
YawErr1 = UserYaw - Yaw;
YawErrSum = YawErrSum + YawErr1;

pid_p = kp*YawErr1;
pid_i = ki*YawErrSum;
pid_d = kd*((YawErr1 - YawErr4)/0.005 + 2*(YawErr2 - YawErr3)/0.005);

PitchOutTerm = pid_p + pid_i + pid_d; %단위: rad(라디안은 무차원임)
%PitchOutTerm = PrevPidOut + pid_p + pid_i + pid_d;
end
